simulink model "zadp_twin"  (R2026a)
settings: Solver=FixedStepDiscrete  StopTime=600  FixedStep=0.02
PreLoadFcn:
  | if isempty(which('BrainSystem')), run('E:\catrover_dumpautonomy\twin3d\startup.m'); end
InitFcn:
  | if isempty(which('BrainSystem')), run('E:\catrover_dumpautonomy\twin3d\startup.m'); end
Description:
  | ZADP hardware digital twin: 3 robots (haul trucks at 1:200) fill the dump plan; 3D view of the run.
settings Model: Creator=richs  LastModifiedBy=richs

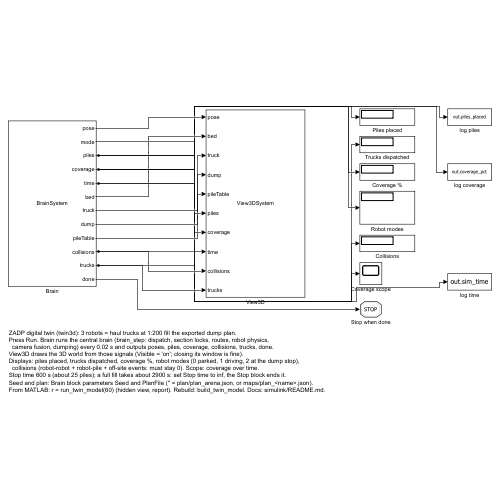
[thumbnail: Simulink's stored preview of the top-level diagram]
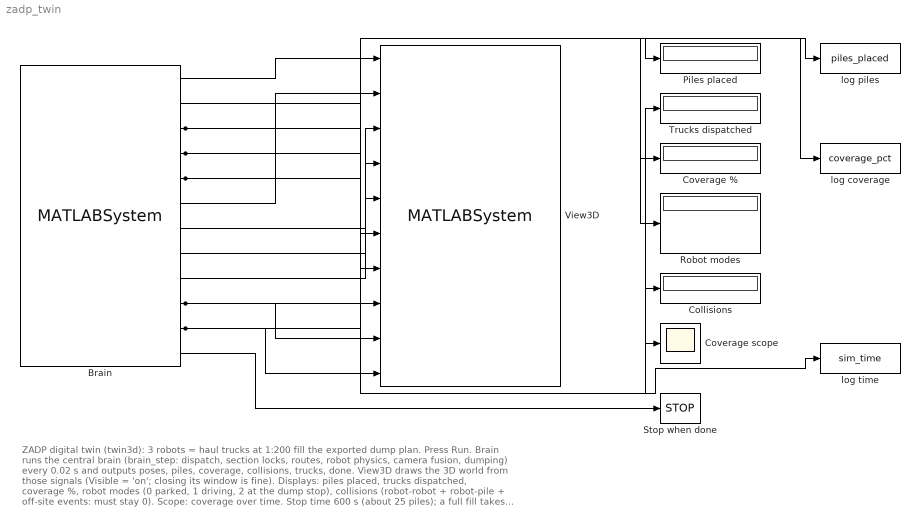
== system zadp_twin ==
  note: ZADP digital twin (twin3d): 3 robots = haul trucks at 1:200 fill the exported dump plan.
      | Press Run. Brain runs the central brain (brain_step: dispatch, section locks, routes, robot physics,
      |   camera fusion, dumping) every 0.02 s and outputs poses, piles, coverage, collisions, trucks, done.
      | View3D draws the 3D world from those signals (Visible = 'on'; closing its window is fine).
      | Displays: piles placed, trucks dispatched, coverage %, robot modes (0 parked, 1 driving, 2 at the dump stop),
      |   collisions (robot-robot + robot-pile + off-site events: must stay 0). Scope: coverage over time.
      | Stop time 600 s (about 25 piles); a full fill takes about 2900 s: set Stop time to inf, the Stop block ends it.
      | Seed and plan: Brain block parameters Seed and PlanFile ('' = plan/plan_arena.json, or maps/plan_<name>.json).
      | From MATLAB: r = run_twin_model(60) (hidden view, report). Rebuild: build_twin_model. Docs: simulink/README.md.
  Brain : MATLABSystem  System=BrainSystem  Seed=1  MaxPiles=130  SampleTime=0.02  SimulateUsing=Interpreted execution
      mask Type: BrainSystem
  Collisions : Display
  Coverage % : Display
  Coverage scope : Scope
  Piles placed : Display
  Robot modes : Display
  Stop when done : Stop
  Trucks dispatched : Display
  View3D : MATLABSystem  System=View3DSystem  Visible=on  RenderPeriod=0.25  SampleTime=0.02  ViewMode=orbit  SimulateUsing=Interpreted execution
      mask Type: View3DSystem
  log coverage : ToWorkspace  VariableName=coverage_pct  SampleTime=-1
  log piles : ToWorkspace  VariableName=piles_placed  SampleTime=-1
  log time : ToWorkspace  VariableName=sim_time  SampleTime=-1
  wires:
  Brain/1 -> View3D/1
  Brain/6 -> View3D/2
  Brain/7 -> View3D/3
  Brain/8 -> View3D/4
  Brain/9 -> View3D/5
  Brain/3 -> View3D/6, Piles placed/1, log piles/1
  Brain/4 -> View3D/7, Coverage %/1, Coverage scope/1, log coverage/1
  Brain/5 -> View3D/8, log time/1
  Brain/10 -> View3D/9, Collisions/1
  Brain/11 -> View3D/10, Trucks dispatched/1
  Brain/2 -> Robot modes/1
  Brain/12 -> Stop when done/1
